simulink model "mdl_VD_st2dofSlipAngles_R2025b_SLX"  (R2025b)
settings: Solver=ode4  StartTime=startTime  StopTime=endTime  FixedStep=deltaT  MaxStep=deltaT  RelTol=1e-3  EnableMultiTasking=on
undefined symbols (not defined in the file): parameters, r, U, V
settings Model: Creator=snb10  LastModifiedBy=snb10
settings SolverCC: AlgebraicLoopSolver=TrustRegion
settings DataIOCC: LimitDataPoints=on  SaveFormat=Array  SignalLoggingSaveFormat=ModelDataLogs  SaveOutput=off  SignalLogging=off  DSMLogging=off  SaveTime=off  SignalLoggingName=sigsOut
settings OptimizationCC: InitFltsAndDblsToZero=on  LifeSpan=inf
settings DebuggingCC: SaveWithParameterizedLinksMsg=none  UnderspecifiedInitializationDetection=Classic  MergeDetectMultiDrivingBlocksExec=none  SignalResolutionControl=TryResolveAllWithWarning  MultiTaskDSMMsg=warning  MultiTaskCondExecSysMsg=none  FcnCallInpInsideContextMsg=warning  UnconnectedInputMsg=warning  UnconnectedOutputMsg=warning  UnconnectedLineMsg=warning  StateNameClashWarn=warning  SFUnexpectedBacktrackingDiag=warning  SFNoUnconditionalDefaultTransitionDiag=warning  SFExecutionAtInitializationDiag=none  ArithmeticOperatorsInVariantConditions=warning
settings HardwareCC: ProdBitPerPointer=32.0  ProdBitPerSizeT=32.0  ProdBitPerPtrDiffT=32.0  ProdLargestAtomicFloat=None  ProdIntDivRoundTo=Undefined  ProdEndianess=Unspecified  ProdWordSize=32.0  ProdHWDeviceType=32-bit Generic  TargetUnknown=on
settings ModelReferenceCC: EnableRefExpFcnMdlSchedulingChecks=on  PropagateSignalLabelsOutOfModel=off
settings SFSimCC: SimUseLocalCustomCode=off  CustomCodeUndefinedFunction=UseInterfaceOnly
settings RTWCC: RTWUseLocalCustomCode=off  GPUComputeCapability=3.5  DLArmComputeVersion=19.05
settings CodeAppCC: StateflowObjectComments=on
settings GRTTargetCC: TargetFcnLib=ansi_tfl_tmw.mat  TargetLangStandard=C89/C90 (ANSI)  CombineOutputUpdateFcns=off  GRTInterface=on
settings ConfigComp: CovMetricSettings=dw  CovSaveCumulativeToWorkspaceVar=on  CovSaveSingleToWorkspaceVar=on  CovExternalEMLEnable=off

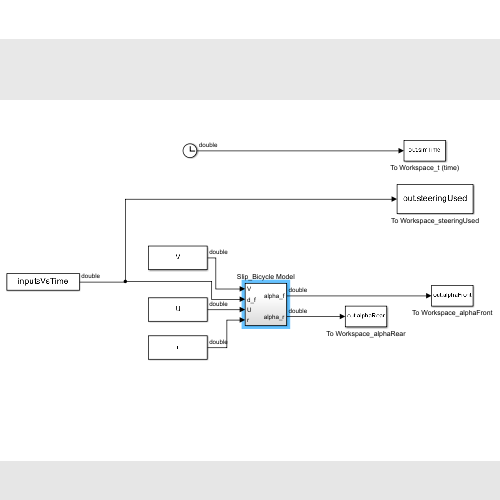
[thumbnail: Simulink's stored preview of the top-level diagram]
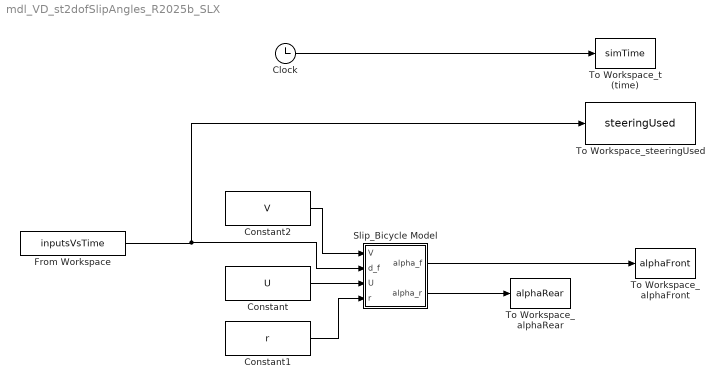
== system mdl_VD_st2dofSlipAngles_R2025b_SLX ==
  Clock : Clock
  Constant : Constant  Value=U  SampleTime=.01
  Constant1 : Constant  Value=r  SampleTime=.01
  Constant2 : Constant  Value=V  SampleTime=.01
  From Workspace : FromWorkspace  VariableName=inputsVsTime  OutDataTypeStr=double  SampleTime=.01  OutputAfterFinalValue=Holding final value
  Slip_Bicycle Model : Subsystem
  To Workspace_alphaFront : ToWorkspace  VariableName=alphaFront  SampleTime=.01
  To Workspace_alphaRear : ToWorkspace  VariableName=alphaRear  SampleTime=.01
  To Workspace_steeringUsed : ToWorkspace  VariableName=steeringUsed  SampleTime=.01
  To Workspace_t (time) : ToWorkspace  VariableName=simTime  SampleTime=.01
  wires:
  Clock/1 -> To Workspace_t (time)/1
  Slip_Bicycle Model/1(alpha_f) -> To Workspace_alphaFront/1
  Slip_Bicycle Model/2(alpha_r) -> To Workspace_alphaRear/1
  From Workspace/1 -> To Workspace_steeringUsed/1, Slip_Bicycle Model/2(d_f)
  Constant/1 -> Slip_Bicycle Model/3(U)
  Constant1/1 -> Slip_Bicycle Model/4(r)
  Constant2/1 -> Slip_Bicycle Model/1(V)

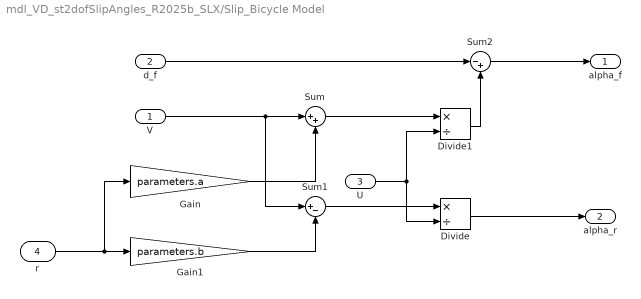
== system mdl_VD_st2dofSlipAngles_R2025b_SLX/Slip_Bicycle Model ==
  V : Inport
  d_f : Inport  Port=2
  U : Inport  Port=3
  r : Inport  Port=4
  Divide : Product  Inputs=*/
  Divide1 : Product  Inputs=*/
  Gain : Gain  Gain=parameters.a
  Gain1 : Gain  Gain=parameters.b
  Sum : Sum  Inputs=|++
  Sum1 : Sum  Inputs=|+-
  Sum2 : Sum  Inputs=|-+
  alpha_f : Outport
  alpha_r : Outport  Port=2
  wires:
  V/1 -> Sum/1, Sum1/1
  Gain/1 -> Sum/2
  r/1 -> Gain/1, Gain1/1
  Gain1/1 -> Sum1/2
  Sum/1 -> Divide1/1
  U/1 -> Divide1/2, Divide/2
  Sum1/1 -> Divide/1
  Divide1/1 -> Sum2/2
  d_f/1 -> Sum2/1
  Sum2/1 -> alpha_f/1
  Divide/1 -> alpha_r/1
